simulink model "sm_car"  (R2025a)
settings: Solver=ode23t  StartTime=0.0  StopTime=400  MaxStep=0.4  RelTol=1e-3  AbsTol=1e-3  EnableMultiTasking=on
PreLoadFcn:
  | % Due to usability issue in Repeating Sequence block
  | warning('off','Simulink:Masking:Invalid');
  | 
  | % Eliminate unnecessary warnings in inactive variants
  | % Warnings generated only if you click through inactive variant
  | warning('off','MATLAB:nonExistentField');
  | warning('off','Simulink:Parameters:BlkParamUndefined');
PostLoadFcn:
  | set_param([bdroot '/Vehicle'],'popup_trailer','Off')
  | warning('off','sm:sli:setup:compile:LocalSolverNotSupported')
  | %sm_car_config_maneuver(bdroot,'WOT Braking');
  | sm_car_config_vehicle(bdroot,'false');
  | sm_car_config_logging(bdroot);
InitFcn:
  | sm_car_config_camera;
  | Vehicle = sm_car_vehcfg_checkConfig(Vehicle);
  | sm_car_check_tire_model(bdroot);
StartFcn:
  | tic;
StopFcn:
  | Elapsed_Sim_Time = toc;
  | % disp(['Elapsed Sim Time = ' num2str(Elapsed_Sim_Time)]);
undefined symbols (not defined in the file): Axle1D, AxleIn, Camera, Control, Driver, Free, Init, Maneuver, Pedal, RaceFix, RaceSpin, Scene, ShaftL1, ShaftL2, ShaftR1, ShaftR2, Soft, Stiff, Visual, X, xy_data_car_side, Y, Z
libraries: sm_lib x1546, nesl_utility x528, fl_lib x480, SimscapeFluids_lib x61, sdl_lib x49, simulink x29, ee_lib x7, simulink_extras x6, Linkage_Systems x4, Tire_1x2x x4, AntiRollBar_Systems x2, Linkage_Decoupled x2
(part 17 of 79)

== system sm_car/Vehicle/Vehicle/Chassis/Spring/Decoupled/Spring A1 Heave ==
  "Ctrl " : Inport
  AirOilPiston : Subsystem  VariantControl=AirOilPiston  mask(Hydropneumatic Spring Damper with Ride Height Control){spr_hp_top=Spring.sTop.Value, spr_hp_bot=Spring.sBottom.Value, t_ambient=Spring.Spring.TAmbient.Value, gspr_gas_properties=Spring.Spring.GasProperties, strut_oil_properties=Spring.Strut.OilProperties, gas_chamber_soft_area=Spring.Spring.GasSoft.A.Value, gas_chamber_stiff_area=Spring.Spring.GasStiff.A.Value, gas_chamber_soft_deadvol=Spring.Spring.GasSoft.volDead.Value, gas_chamber_stiff_deadvol=Spring.Spring.GasStiff.volDead.Value, gspr_mass_soft=Spring.Spring.GasSoft.mPiston.Value, gspr_mass_stiff=Spring.Spring.GasStiff.mPiston.Value, gspr_damping_soft=Spring.Spring.GasSoft.b.Value, gspr_damping_stiff=Spring.Spring.GasStiff.b.Value, gas_chamber_soft_x0=Spring.Spring.GasSoft.xInit.Value, gas_chamber_stiff_x0=Spring.Spring.GasStiff.xInit.Value, gas_chamber_soft_p0=Spring.Spring.GasSoft.pInit.Value, gas_chamber_stiff_p0=Spring.Spring.GasStiff.pInit.Value, gspr_cwall_soft=Spring.Spring.GasSoft.CWall.Value, gspr_cwall_stiff=Spring.Spring.GasStiff.CWall.Value, oil_chamber_soft_area=Spring.Spring.OilSoft.A.Value, oil_chamber_stiff_area=Spring.Spring.OilStiff.A.Value, oil_chamber_soft_deadvol=Spring.Spring.OilSoft.volDead.Value, oil_chamber_stiff_deadvol=Spring.Spring.OilStiff.volDead.Value, oil_chamber_soft_x0=Spring.Spring.OilSoft.xInit.Value, oil_chamber_stiff_x0=Spring.Spring.OilStiff.xInit.Value, oil_chamber_soft_p0=Spring.Spring.OilSoft.pInit.Value, oil_chamber_stiff_p0=Spring.Spring.OilStiff.pInit.Value, gsprv_smax_soft=Spring.Spring.ValveSoft.xMaxOpen.Value, gsprv_smax_stiff=Spring.Spring.ValveStiff.xMaxOpen.Value, gsprv_delsmax_soft=Spring.Spring.ValveSoft.xCloseToOpen.Value, gsprv_delsmax_stiff=Spring.Spring.ValveStiff.xCloseToOpen.Value, gsprv_arealeak_soft=Spring.Spring.ValveSoft.areaLeak.Value, gsprv_arealeak_stiff=Spring.Spring.ValveStiff.areaLeak.Value, gsprv_areamax_soft=Spring.Spring.ValveSoft.aMax.Value, gsprv_areamax_stiff=Spring.Spring.ValveStiff.aMax.Value, gsprv_cd_soft=Spring.Spring.ValveSoft.Cd.Value, gsprv_cd_stiff=Spring.Spring.ValveStiff.Cd.Value, gsprv_smooth_soft=Spring.Spring.ValveSoft.smoothFactor.Value, gsprv_smooth_stiff=Spring.Spring.ValveStiff.smoothFactor.Value, gsprva_stroke_soft=Spring.Spring.ValveActuatorSoft.xStroke.Value, gsprva_stroke_stiff=Spring.Spring.ValveActuatorStiff.xStroke.Value, gsprva_ton_soft=Spring.Spring.ValveActuatorSoft.tOn.Value, gsprva_ton_stiff=Spring.Spring.ValveActuatorStiff.tOn.Value, gsprva_toff_soft=Spring.Spring.ValveActuatorSoft.tOff.Value, gsprva_toff_stiff=Spring.Spring.ValveActuatorStiff.tOff.Value, strut_deadvol=Spring.Strut.volDead.Value, strut_area=Spring.Strut.A.Value, strut_x0=Spring.Strut.xInit.Value, strut_frc_colfrc=Spring.Strut.Friction.fCoulomb.Value, strut_frc_brkfrc=Spring.Strut.Friction.fBreakaway.Value, strut_frc_brkvel=Spring.Strut.Friction.vBreakaway.Value, strut_frc_visccoeff=Spring.Strut.Friction.mu.Value, bs_lim_upper=Spring.Endstop.xMax.Value, bs_lim_lower=Spring.Endstop.xMin.Value, bs_k_upper=Spring.Endstop.KxMax.Value, bs_k_lower=Spring.Endstop.KxMin.Value, bs_b_upper=Spring.Endstop.dxMax.Value, bs_b_lower=Spring.Endstop.dxMin.Value, bs_region=Spring.Endstop.xTransition.Value, p_diff_TLU_constant=Spring.Damper.Orifice.pDiff.Value, vol_flow_TLU_constant=Spring.Damper.Orifice.q.Value, dpr_restrarea_comp=Spring.Damper.RestrictionComp.A.Value, dpr_restrarea_reb=Spring.Damper.RestrictionReb.A.Value, dpr_cd_comp=Spring.Damper.RestrictionComp.Cd.Value, dpr_cd_reb=Spring.Damper.RestrictionReb.Cd.Value, dpr_prv_psetdiff_comp=Spring.Damper.PRVComp.pDiff.Value, dpr_prv_psetdiff_reb=Spring.Damper.PRVReb.pDiff.Value, dpr_prv_prange_comp=Spring.Damper.PRVComp.pRange.Value, dpr_prv_prange_reb=Spring.Damper.PRVReb.pRange.Value, dpr_prv_areamax_comp=Spring.Damper.PRVComp.A.Value, dpr_prv_areamax_reb=Spring.Damper.PRVReb.A.Value, dpr_prv_cd_comp=Spring.Damper.PRVComp.Cd.Value, dpr_prv_cd_reb=Spring.Damper.PRVReb.Cd.Value, dpr_cvdvalve_cmpos=Spring.CVDValve.Orifice.x.Value, dpr_cvdvalve_orifice_area=Spring.CVDValve.Orifice.A.Value, dpr_cvdvalve_orifice_pdiff=Spring.CVDValve.Orifice.pDiff.Value, dpr_cvdvalve_pcv_areamax=Spring.CVDValve.PCValve.AMax.Value, dpr_cvdvalve_pcv_prange=Spring.CVDValve.PCValve.pRange.Value, dpr_cvdvalve_arealeak=Spring.CVDValve.PCValve.ALeak.Value, dpr_cvdvalve_cd=Spring.CVDValve.PCValve.Cd.Value, dpr_cvdvalve_act_ts=Spring.CVDValve.tFilt.Value, rh_srcpressure=Spring.RideHeight.pSource.Value, rh_fcv_cmpos_inlet=Spring.RideHeight.OrificeInlet.x.Value, rh_fcv_cmpos_outlet=Spring.RideHeight.OrificeOutlet.x.Value, rh_fcv_orificearea_inlet=Spring.RideHeight.OrificeInlet.A.Value, rh_fcv_orificearea_outlet=Spring.RideHeight.OrificeOutlet.A.Value, rh_fcv_orificepdiff_inlet=Spring.RideHeight.OrificeInlet.pDiff.Value, rh_fcv_orificepdiff_outlet=Spring.RideHeight.OrificeOutlet.pDiff.Value, rh_fcv_pcprange_inlet=Spring.RideHeight.PCValveInlet.pRange.Value, rh_fcv_pcprange_outlet=Spring.RideHeight.PCValveOutlet.pRange.Value, rh_fcv_pcamax_inlet=Spring.RideHeight.PCValveInlet.AMax.Value, rh_fcv_pcamax_outlet=Spring.RideHeight.PCValveOutlet.AMax.Value, rh_fcv_arealeak_inlet=Spring.RideHeight.PCValveInlet.ALeak.Value, rh_fcv_arealeak_outlet=Spring.RideHeight.PCValveOutlet.ALeak.Value, rh_fcv_cd_inlet=Spring.RideHeight.PCValveInlet.Cd.Value, rh_fcv_cd_outlet=Spring.RideHeight.PCValveOutlet.Cd.Value, rh_fcv_smooth_inlet=Spring.RideHeight.PCValveInlet.smoothFactor.Value, rh_fcv_smooth_outlet=Spring.RideHeight.PCValveOutlet.smoothFactor.Value, rh_fcv_tfilt_inlet=Spring.RideHeight.PCValveInlet.tFilt.Value, rh_fcv_tfilt_outlet=Spring.RideHeight.PCValveOutlet.tFilt.Value}
      mask prompts: spr_hp_top "HP Top (m)"; spr_hp_bot "HP Bottom (m)"; t_ambient "Ambient Temperature (K)"; gspr_gas_properties "Gas Properties"; strut_oil_properties "Oil Properties"; strut_deadvol "Dead Volume (l)"; strut_area "Area (m^2)"; strut_x0 "Initial Disp. (m)"; strut_frc_colfrc "Coulomb Friction (N)"; strut_frc_brkfrc "Breakaway Force (N)"; strut_frc_brkvel "Breakaway Vel (m/s)"; strut_frc_visccoeff "Viscous Friction (N/(m/s))"; bs_region "Transition Region (m)"; p_diff_TLU_constant "Pressure Drop Vector (MPa)"; vol_flow_TLU_constant "Vol Flow Rate (m^3/s)"; dpr_cvdvalve_cmpos "Orifice Pos. Vector (m)"; dpr_cvdvalve_orifice_area "Orifice Area (m^2)"; dpr_cvdvalve_orifice_pdiff "Orifice Set Press. Diff. (bar)"; dpr_cvdvalve_pcv_areamax "Pr. Comp. Valve Max Area (m^2)"; dpr_cvdvalve_pcv_prange "Pr. Comp. Valve Range (bar)"; dpr_cvdvalve_arealeak "Leakage Area (m^2)"; dpr_cvdvalve_cd "Discharge Coeff (Cd)"; dpr_cvdvalve_act_ts "Actuator Time Constant (s)"; rh_srcpressure "Source Pressure (MPa)"
      mask help: Hydropneumatic spring damper with ride height control. Control signal selects soft or stiff gas spring. Damper has unique rebound and compression characteristics. Ride height can be raised or lowered.
      mask init:
      | spr_len0 = norm(spr_hp_top-spr_hp_bot);
      | 
      | gasprop_R  = gspr_gas_properties.R.Value;
      | gasprop_h  = gspr_gas_properties.h.Value;
      | gasprop_cp = gspr_gas_properties.cp.Value;
      | gasprop_mu = gspr_gas_properties.mu.Value;
      | gasprop_k  = gspr_gas_properties.k.Value;
      | 
      | oilprop_rho = strut_oil_properties.rho.Value;
      | oilprop_B   = strut_oil_properties.B.Value;
      | oilprop_nu  = strut_oil_properties.nu.Value;
      mask TypeOptions t_ambient: Ambient/temperature
      mask TypeOptions gas_chamber_soft_area:
      | Chamber
      | Gas Spring
      | Soft/interface_area
      mask TypeOptions gas_chamber_stiff_area:
      | Chamber
      | Gas Spring
      | Stiff/interface_area
      mask TypeOptions gas_chamber_soft_deadvol:
      | Chamber
      | Gas Spring
      | Soft/dead_volume
      mask TypeOptions gas_chamber_stiff_deadvol:
      | Chamber
      | Gas Spring
      | Stiff/dead_volume
      mask TypeOptions gspr_mass_soft:
      | Mass
      | Gas Spring
      | Soft/mass
      mask TypeOptions gspr_mass_stiff:
      | Mass
      | Gas Spring
      | Stiff/mass
      mask TypeOptions gspr_damping_soft:
      | Damper
      | Gas
      | Spring
      | Soft/D
      mask TypeOptions gspr_damping_stiff:
      | Damper
      | Gas
      | Spring
      | Stiff
      | /D
      mask TypeOptions gas_chamber_soft_x0:
      | Chamber
      | Gas Spring
      | Soft/length_init
      mask TypeOptions gas_chamber_stiff_x0:
      | Chamber
      | Gas Spring
      | Stiff/length_init
      mask TypeOptions gas_chamber_soft_p0:
      | Chamber
      | Gas Spring
      | Soft/p_I
      mask TypeOptions gas_chamber_stiff_p0:
      | Chamber
      | Gas Spring
      | Stiff/p_I
      mask TypeOptions gspr_cwall_soft: ThermResGasSoft/resistance
      mask TypeOptions gspr_cwall_stiff: ThermResGasStiff/resistance
      mask TypeOptions oil_chamber_soft_area:
      | Chamber
      | Oil Soft/interface_area
      mask TypeOptions oil_chamber_stiff_area:
      | Chamber
      | Oil Stiff/interface_area
      mask TypeOptions oil_chamber_soft_deadvol:
      | Chamber
      | Oil Soft/dead_volume
      mask TypeOptions oil_chamber_stiff_deadvol:
      | Chamber
      | Oil Stiff/dead_volume
      mask TypeOptions oil_chamber_soft_x0:
      | Chamber
      | Oil Soft/x0
      mask TypeOptions oil_chamber_stiff_x0:
      | Chamber
      | Oil Stiff/x0
      mask TypeOptions oil_chamber_soft_p0:
      | Chamber
      | Oil Soft/p0
      mask TypeOptions oil_chamber_stiff_p0:
      | Chamber
      | Oil Stiff/p0
      mask TypeOptions gsprv_smax_soft:
      | Valve Soft
      | SV10-24 NC/S_max
      mask TypeOptions gsprv_smax_stiff:
      | Valve Stiff
      | SV10-25 NO/S_max
      mask TypeOptions gsprv_delsmax_soft:
      | Valve Soft
      | SV10-24 NC/del_S_max
      mask TypeOptions gsprv_delsmax_stiff:
      | Valve Stiff
      | SV10-25 NO/del_S_max
      mask TypeOptions gsprv_arealeak_soft:
      | Valve Soft
      | SV10-24 NC/area_leak
      mask TypeOptions gsprv_arealeak_stiff:
      | Valve Stiff
      | SV10-25 NO/area_leak
      mask TypeOptions gsprv_areamax_soft:
      | Valve Soft
      | SV10-24 NC/area_max
      mask TypeOptions gsprv_areamax_stiff:
      | Valve Stiff
      | SV10-25 NO/area_max
      mask TypeOptions gsprv_cd_soft:
      | Valve Soft
      | SV10-24 NC/Cd
      mask TypeOptions gsprv_cd_stiff:
      | Valve Stiff
      | SV10-25 NO/Cd
      mask TypeOptions gsprv_smooth_soft:
      | Valve Soft
      | SV10-24 NC/smoothing_factor
      mask TypeOptions gsprv_smooth_stiff:
      | Valve Stiff
      | SV10-25 NO/smoothing_factor
      mask TypeOptions gsprva_stroke_soft:
      | Valve Actuator
      | Spring Soft/stroke
      mask TypeOptions gsprva_stroke_stiff:
      | Valve Actuator
      | Spring Stiff/stroke
      mask TypeOptions gsprva_ton_soft:
      | Valve Actuator
      | Spring Soft/t_on
      mask TypeOptions gsprva_ton_stiff:
      | Valve Actuator
      | Spring Stiff/t_on
      mask TypeOptions gsprva_toff_soft:
      | Valve Actuator
      | Spring Soft/t_off
      mask TypeOptions gsprva_toff_stiff:
      | Valve Actuator
      | Spring Stiff/t_off
      mask TypeOptions strut_deadvol:
      | Chamber
      | Strut/dead_volume
      mask TypeOptions strut_area:
      | Chamber
      | Strut/interface_area
      mask TypeOptions strut_x0:
      | Chamber
      | Strut/x0
      mask TypeOptions strut_frc_colfrc:
      | Strut
      | Friction/Col_frc
      mask TypeOptions strut_frc_brkfrc:
      | Strut
      | Friction/brkwy_frc
      mask TypeOptions strut_frc_brkvel:
      | Strut
      | Friction/brkwy_vel
      mask TypeOptions strut_frc_visccoeff:
      | Strut
      | Friction/visc_coef
      mask TypeOptions bs_lim_upper:
      | Strut
      | Hard
      | Stop/upper_bnd
      mask TypeOptions bs_lim_lower:
      | Strut
      | Hard
      | Stop/lower_bnd
      mask TypeOptions bs_k_upper:
      | Strut
      | Hard
      | Stop/stiff_up
      mask TypeOptions bs_k_lower:
      | Strut
      | Hard
      | Stop/stiff_low
      mask TypeOptions bs_b_upper:
      | Strut
      | Hard
      | Stop/D_up
      mask TypeOptions bs_b_lower:
      | Strut
      | Hard
      | Stop/D_low
      mask TypeOptions bs_region:
      | Strut
      | Hard
      | Stop/transition
      mask TypeOptions p_diff_TLU_constant: Damper/p_diff_TLU_constant
      mask TypeOptions vol_flow_TLU_constant: Damper/vol_flow_TLU_constant
      mask TypeOptions dpr_restrarea_comp: Damper/dpr_restrarea_comp
      mask TypeOptions dpr_restrarea_reb: Damper/dpr_restrarea_reb
      mask TypeOptions dpr_cd_comp: Damper/dpr_cd_comp
      mask TypeOptions dpr_cd_reb: Damper/dpr_cd_reb
      mask TypeOptions dpr_prv_psetdiff_comp: Damper/dpr_prv_psetdiff_comp
      mask TypeOptions dpr_prv_psetdiff_reb: Damper/dpr_prv_psetdiff_reb
      mask TypeOptions dpr_prv_prange_comp: Damper/dpr_prv_prange_comp
      mask TypeOptions dpr_prv_prange_reb: Damper/dpr_prv_prange_reb
      mask TypeOptions dpr_prv_areamax_comp: Damper/dpr_prv_areamax_comp
      mask TypeOptions dpr_prv_areamax_reb: Damper/dpr_prv_areamax_reb
      mask TypeOptions dpr_prv_cd_comp: Damper/dpr_prv_cd_comp
      mask TypeOptions dpr_prv_cd_reb: Damper/dpr_prv_cd_reb
      mask TypeOptions dpr_cvdvalve_cmpos: Damper/dpr_cvdvalve_cmpos
      mask TypeOptions dpr_cvdvalve_orifice_area: Damper/dpr_cvdvalve_orifice_area
      mask TypeOptions dpr_cvdvalve_orifice_pdiff: Damper/dpr_cvdvalve_orifice_pdiff
      mask TypeOptions dpr_cvdvalve_pcv_areamax: Damper/dpr_cvdvalve_pcv_areamax
      mask TypeOptions dpr_cvdvalve_pcv_prange: Damper/dpr_cvdvalve_pcv_prange
      mask TypeOptions dpr_cvdvalve_arealeak: Damper/dpr_cvdvalve_arealeak
      mask TypeOptions dpr_cvdvalve_cd: Damper/dpr_cvdvalve_cd
      mask TypeOptions dpr_cvdvalve_act_ts: Damper/dpr_cvdvalve_act_ts
      mask TypeOptions rh_srcpressure: Ride Height/rh_srcpressure
      mask TypeOptions rh_fcv_cmpos_inlet: Ride Height/rh_fcv_cmpos_inlet
      mask TypeOptions rh_fcv_cmpos_outlet: Ride Height/rh_fcv_cmpos_outlet
      mask TypeOptions rh_fcv_orificearea_inlet: Ride Height/rh_fcv_orificearea_inlet
      mask TypeOptions rh_fcv_orificearea_outlet: Ride Height/rh_fcv_orificearea_outlet
      mask TypeOptions rh_fcv_orificepdiff_inlet: Ride Height/rh_fcv_orificepdiff_inlet
      mask TypeOptions rh_fcv_orificepdiff_outlet: Ride Height/rh_fcv_orificepdiff_outlet
      mask TypeOptions rh_fcv_pcprange_inlet: Ride Height/rh_fcv_pcprange_inlet
      mask TypeOptions rh_fcv_pcprange_outlet: Ride Height/rh_fcv_pcprange_outlet
      mask TypeOptions rh_fcv_pcamax_inlet: Ride Height/rh_fcv_pcamax_inlet
      mask TypeOptions rh_fcv_pcamax_outlet: Ride Height/rh_fcv_pcamax_outlet
      mask TypeOptions rh_fcv_arealeak_inlet: Ride Height/rh_fcv_arealeak_inlet
      mask TypeOptions rh_fcv_arealeak_outlet: Ride Height/rh_fcv_arealeak_outlet
      mask TypeOptions rh_fcv_cd_inlet: Ride Height/rh_fcv_cd_inlet
      mask TypeOptions rh_fcv_cd_outlet: Ride Height/rh_fcv_cd_outlet
      mask TypeOptions rh_fcv_smooth_inlet: Ride Height/rh_fcv_smooth_inlet
      mask TypeOptions rh_fcv_smooth_outlet: Ride Height/rh_fcv_smooth_outlet
      mask TypeOptions rh_fcv_tfilt_inlet: Ride Height/rh_fcv_tfilt_inlet
      mask TypeOptions rh_fcv_tfilt_outlet: Ride Height/rh_fcv_tfilt_outlet
      mask DialogControl tab_gas_spring Prompt: Gas Spring
      mask DialogControl cont_gas_spring_gas Prompt: Gas Side
      mask DialogControl text_gspr_soft Prompt: Soft
      mask DialogControl text_gspr_stiff Prompt: Stiff
      mask DialogControl text_gspr_area Prompt: Area (m^2)
      mask DialogControl text_gspr_deadvol Prompt: Dead Volume (l)
      mask DialogControl text_gspr_pistmass Prompt: Piston Mass (kg)
      mask DialogControl text_gspr_damping Prompt: Damping (N/(m/s))
      mask DialogControl text_gspr_x0 Prompt: Initial Disp. (m)
      mask DialogControl text_gspr_p0 Prompt: Initial Press. (MPa)
      mask DialogControl text_gspr_cwall Prompt: Wall (K/W)
      mask DialogControl cont_gas_spring_oil Prompt: Oil Side
      mask DialogControl text_gspro_soft Prompt: Soft
      mask DialogControl text_gspro_stiff Prompt: Stiff
      mask DialogControl text_gspro_area Prompt: Area (m^2)
      mask DialogControl text_gspro_deadvol Prompt: Dead Volume (l)
      mask DialogControl text_gspro_x0 Prompt: Initial Disp. (m)
      mask DialogControl text_oil_chamber_x0 Prompt: Initial Press. (MPa)
      mask DialogControl cont_gas_spring_valve Prompt: Valve
      mask DialogControl text_gsprv_soft Prompt: Soft
      mask DialogControl text_gsprv_stiff Prompt: Stiff
      mask DialogControl text_gsprv_xopen Prompt: Travel at Open (m)
      mask DialogControl text_gsprv_delSmax Prompt: Closed to Open (m)
      mask DialogControl text_gsprv_areaLeak Prompt: Leakage (m^2)
      mask DialogControl text_gsprv_areaMax Prompt: Area Max (m^2)
      mask DialogControl text_gsprv_cd Prompt: Cd
      mask DialogControl text_gsprv_smooth Prompt: Smooth
      mask DialogControl cont_gas_spring_valveact Prompt: Valve Actuator
      mask DialogControl text_gsprva_soft Prompt: Soft
      mask DialogControl text_gsprva_stiff Prompt: Stiff
      mask DialogControl text_gsprva_stroke Prompt: Stroke (m)
      mask DialogControl text_gsprva_ton Prompt: On Time (s)
      mask DialogControl text_gsprva_toff Prompt: Off Time (s)
      mask DialogControl cont_oil_strut Prompt: Strut
      mask DialogControl cont_endstop Prompt: Endstop
      mask DialogControl text_endstop_upper Prompt: Upper
      mask DialogControl text_endstop_lower Prompt: Lower
      mask DialogControl text_endstop_limit Prompt: Limit (m)
      mask DialogControl text_endstop_stiffness Prompt: Stiffness (N/m)
      mask DialogControl text_endstop_damping Prompt: Damping (N/(m/s))
      mask DialogControl tab_damper Prompt: Damper
      mask DialogControl cont_orifice_ls Prompt: Low Speed Orifice
      mask DialogControl cont_blowoff_restriction Prompt: Blowoff Restriction
      mask DialogControl text_blowoff_comp Prompt: Compression
      mask DialogControl text_blowoff_reb Prompt: Rebound
      mask DialogControl text_restr_area Prompt: Restr. Area (m^2)
      mask DialogControl text_cd Prompt: Cd
      mask DialogControl cont_blowoff_prv Prompt: Blowoff PRV
      mask DialogControl text_blowoff_prv_comp Prompt: Compression
      mask DialogControl text_blowoff_prv_reb Prompt: Rebound
      mask DialogControl text_psetdiff Prompt: Press. Diff. (MPa)
      mask DialogControl text_prange Prompt: Press. Range (MPa)
      mask DialogControl text_areamax Prompt: Max Area (m^2)
      mask DialogControl text_blowoff_cd Prompt: Cd
      mask DialogControl cont_dpr_cvd_valve Prompt: CVD Valve
      mask DialogControl tab_ride_height Prompt: Ride Height
      mask DialogControl text_rideheight_inlet Prompt: Inlet
      mask DialogControl text_rideheight_outlet Prompt: Outlet
      mask DialogControl text_rh_prcv_cmpos Prompt: Orifice Pos. Vec. (m)
      mask DialogControl text_rh_prcv_orificearea Prompt: Orifice Area Vec (m^2)
      mask DialogControl text_rh_prcv_orificepdiff Prompt: Orifice Pr. Diff (bar)
      mask DialogControl text_rh_prcv_pcprange Prompt: Pr. Comp. Range (bar)
      mask DialogControl text_rh_prcv_pcamax Prompt: Pr. Comp. A Max (m^2)
      mask DialogControl text_rh_prcv_arealeak Prompt: Leakage Area (m^2)
      mask DialogControl text_rh_prcv_cd Prompt: Cd
      mask DialogControl text_rh_fcv_smooth Prompt: Smoothing
      mask DialogControl text_rh_fcv_tfilt Prompt: Time Constant (s)
  Linear : Subsystem  VariantControl=Linear  mask(Linear Spring){spr_def0=Spring.xPreload.Value, spr_frc0=Spring.fPreload.Value, spr_k=Spring.K.Value, spr_hp_top=Spring.sTop.Value, spr_hp_bot=Spring.sBottom.Value}
      mask prompts: spr_def0 "Preload Deformation (m)"; spr_frc0 "Preload Force (N)"; spr_k "Spring Rate (N/m)"; spr_hp_top "HP Top [xyz] (m)"; spr_hp_bot "HP Bottom [xyz] (m)"
      mask help: Spring with linear stiffness. Preload can be specified using deformation or force, unused value must be zero. If both are non-zero, preload deformation is used.
      mask init:
      | spr_len0 = norm(spr_hp_top-spr_hp_bot);
      | 
      | curblk = gcb;
      | if(abs(spr_def0)>0)
      | set_param([curblk '/Spring'],...
      |     'f_specify','Off',...
      |     'x_priority','High');
      | else
      | set_param([curblk '/Spring'],...
      |     'f_specify','On',...
      |     'x_priority','None');
      | end
      mask DialogControl Container3 Prompt: Specify Preload Deformation or Force, other value is 0
  No Spring : Subsystem  VariantControl=No_Spring  mask(No Spring){}
      mask help: Sensor only
  Nonlinear : Subsystem  VariantControl=Nonlinear  mask(Nonlinear Spring){spr_def0=Spring.xPreload.Value, spr_frc0=Spring.fPreload.Value, deformation_vector=Spring.xSpring.Value, force_vector=Spring.fSpring.Value, spr_hp_top=Spring.sTop.Value, spr_hp_bot=Spring.sBottom.Value}
      mask prompts: spr_def0 "Preload Deformation (m)"; spr_frc0 "Preload Force (N)"; deformation_vector "Deformation vector"; force_vector "Force vector"; spr_hp_top "HP Top [xyz] (m)"; spr_hp_bot "HP Bottom [xyz] (m)"
      mask help: Spring with stiffness specified by a lookup table. Preload can be specified using deformation or force, unused value must be zero. If both are non-zero, preload deformation is used.
      mask init:
      | spr_len0 = norm(spr_hp_top-spr_hp_bot);
      | 
      | curblk = gcb;
      | spr_x0 = -spr_def0;
      | if(spr_def0==0 && (abs(spr_frc0)>0))
      | spr_x0 = -interp1(force_vector,deformation_vector,spr_frc0);
      | end
      mask TypeOptions deformation_vector: Spring/deformation_vector
      mask TypeOptions force_vector: Spring/force_vector
      mask DialogControl Container3 Prompt: Specify Preload Deformation or Force, other value is 0
  " R" : PMIOPort  Side=Left
  " C" : PMIOPort  Port=2  Side=Right
  " meas" : Outport  VectorParamsAs1DForOutWhenUnconnected=off

== system sm_car/Vehicle/Vehicle/Chassis/Spring/Decoupled/Spring A1 Roll ==
  "Ctrl " : Inport
  AirOilPiston : Subsystem  VariantControl=AirOilPiston  mask(Hydropneumatic Spring Damper with Ride Height Control){spr_hp_top=Spring.sTop.Value, spr_hp_bot=Spring.sBottom.Value, t_ambient=Spring.Spring.TAmbient.Value, gspr_gas_properties=Spring.Spring.GasProperties, strut_oil_properties=Spring.Strut.OilProperties, gas_chamber_soft_area=Spring.Spring.GasSoft.A.Value, gas_chamber_stiff_area=Spring.Spring.GasStiff.A.Value, gas_chamber_soft_deadvol=Spring.Spring.GasSoft.volDead.Value, gas_chamber_stiff_deadvol=Spring.Spring.GasStiff.volDead.Value, gspr_mass_soft=Spring.Spring.GasSoft.mPiston.Value, gspr_mass_stiff=Spring.Spring.GasStiff.mPiston.Value, gspr_damping_soft=Spring.Spring.GasSoft.b.Value, gspr_damping_stiff=Spring.Spring.GasStiff.b.Value, gas_chamber_soft_x0=Spring.Spring.GasSoft.xInit.Value, gas_chamber_stiff_x0=Spring.Spring.GasStiff.xInit.Value, gas_chamber_soft_p0=Spring.Spring.GasSoft.pInit.Value, gas_chamber_stiff_p0=Spring.Spring.GasStiff.pInit.Value, gspr_cwall_soft=Spring.Spring.GasSoft.CWall.Value, gspr_cwall_stiff=Spring.Spring.GasStiff.CWall.Value, oil_chamber_soft_area=Spring.Spring.OilSoft.A.Value, oil_chamber_stiff_area=Spring.Spring.OilStiff.A.Value, oil_chamber_soft_deadvol=Spring.Spring.OilSoft.volDead.Value, oil_chamber_stiff_deadvol=Spring.Spring.OilStiff.volDead.Value, oil_chamber_soft_x0=Spring.Spring.OilSoft.xInit.Value, oil_chamber_stiff_x0=Spring.Spring.OilStiff.xInit.Value, oil_chamber_soft_p0=Spring.Spring.OilSoft.pInit.Value, oil_chamber_stiff_p0=Spring.Spring.OilStiff.pInit.Value, gsprv_smax_soft=Spring.Spring.ValveSoft.xMaxOpen.Value, gsprv_smax_stiff=Spring.Spring.ValveStiff.xMaxOpen.Value, gsprv_delsmax_soft=Spring.Spring.ValveSoft.xCloseToOpen.Value, gsprv_delsmax_stiff=Spring.Spring.ValveStiff.xCloseToOpen.Value, gsprv_arealeak_soft=Spring.Spring.ValveSoft.areaLeak.Value, gsprv_arealeak_stiff=Spring.Spring.ValveStiff.areaLeak.Value, gsprv_areamax_soft=Spring.Spring.ValveSoft.aMax.Value, gsprv_areamax_stiff=Spring.Spring.ValveStiff.aMax.Value, gsprv_cd_soft=Spring.Spring.ValveSoft.Cd.Value, gsprv_cd_stiff=Spring.Spring.ValveStiff.Cd.Value, gsprv_smooth_soft=Spring.Spring.ValveSoft.smoothFactor.Value, gsprv_smooth_stiff=Spring.Spring.ValveStiff.smoothFactor.Value, gsprva_stroke_soft=Spring.Spring.ValveActuatorSoft.xStroke.Value, gsprva_stroke_stiff=Spring.Spring.ValveActuatorStiff.xStroke.Value, gsprva_ton_soft=Spring.Spring.ValveActuatorSoft.tOn.Value, gsprva_ton_stiff=Spring.Spring.ValveActuatorStiff.tOn.Value, gsprva_toff_soft=Spring.Spring.ValveActuatorSoft.tOff.Value, gsprva_toff_stiff=Spring.Spring.ValveActuatorStiff.tOff.Value, strut_deadvol=Spring.Strut.volDead.Value, strut_area=Spring.Strut.A.Value, strut_x0=Spring.Strut.xInit.Value, strut_frc_colfrc=Spring.Strut.Friction.fCoulomb.Value, strut_frc_brkfrc=Spring.Strut.Friction.fBreakaway.Value, strut_frc_brkvel=Spring.Strut.Friction.vBreakaway.Value, strut_frc_visccoeff=Spring.Strut.Friction.mu.Value, bs_lim_upper=Spring.Endstop.xMax.Value, bs_lim_lower=Spring.Endstop.xMin.Value, bs_k_upper=Spring.Endstop.KxMax.Value, bs_k_lower=Spring.Endstop.KxMin.Value, bs_b_upper=Spring.Endstop.dxMax.Value, bs_b_lower=Spring.Endstop.dxMin.Value, bs_region=Spring.Endstop.xTransition.Value, p_diff_TLU_constant=Spring.Damper.Orifice.pDiff.Value, vol_flow_TLU_constant=Spring.Damper.Orifice.q.Value, dpr_restrarea_comp=Spring.Damper.RestrictionComp.A.Value, dpr_restrarea_reb=Spring.Damper.RestrictionReb.A.Value, dpr_cd_comp=Spring.Damper.RestrictionComp.Cd.Value, dpr_cd_reb=Spring.Damper.RestrictionReb.Cd.Value, dpr_prv_psetdiff_comp=Spring.Damper.PRVComp.pDiff.Value, dpr_prv_psetdiff_reb=Spring.Damper.PRVReb.pDiff.Value, dpr_prv_prange_comp=Spring.Damper.PRVComp.pRange.Value, dpr_prv_prange_reb=Spring.Damper.PRVReb.pRange.Value, dpr_prv_areamax_comp=Spring.Damper.PRVComp.A.Value, dpr_prv_areamax_reb=Spring.Damper.PRVReb.A.Value, dpr_prv_cd_comp=Spring.Damper.PRVComp.Cd.Value, dpr_prv_cd_reb=Spring.Damper.PRVReb.Cd.Value, dpr_cvdvalve_cmpos=Spring.CVDValve.Orifice.x.Value, dpr_cvdvalve_orifice_area=Spring.CVDValve.Orifice.A.Value, dpr_cvdvalve_orifice_pdiff=Spring.CVDValve.Orifice.pDiff.Value, dpr_cvdvalve_pcv_areamax=Spring.CVDValve.PCValve.AMax.Value, dpr_cvdvalve_pcv_prange=Spring.CVDValve.PCValve.pRange.Value, dpr_cvdvalve_arealeak=Spring.CVDValve.PCValve.ALeak.Value, dpr_cvdvalve_cd=Spring.CVDValve.PCValve.Cd.Value, dpr_cvdvalve_act_ts=Spring.CVDValve.tFilt.Value, rh_srcpressure=Spring.RideHeight.pSource.Value, rh_fcv_cmpos_inlet=Spring.RideHeight.OrificeInlet.x.Value, rh_fcv_cmpos_outlet=Spring.RideHeight.OrificeOutlet.x.Value, rh_fcv_orificearea_inlet=Spring.RideHeight.OrificeInlet.A.Value, rh_fcv_orificearea_outlet=Spring.RideHeight.OrificeOutlet.A.Value, rh_fcv_orificepdiff_inlet=Spring.RideHeight.OrificeInlet.pDiff.Value, rh_fcv_orificepdiff_outlet=Spring.RideHeight.OrificeOutlet.pDiff.Value, rh_fcv_pcprange_inlet=Spring.RideHeight.PCValveInlet.pRange.Value, rh_fcv_pcprange_outlet=Spring.RideHeight.PCValveOutlet.pRange.Value, rh_fcv_pcamax_inlet=Spring.RideHeight.PCValveInlet.AMax.Value, rh_fcv_pcamax_outlet=Spring.RideHeight.PCValveOutlet.AMax.Value, rh_fcv_arealeak_inlet=Spring.RideHeight.PCValveInlet.ALeak.Value, rh_fcv_arealeak_outlet=Spring.RideHeight.PCValveOutlet.ALeak.Value, rh_fcv_cd_inlet=Spring.RideHeight.PCValveInlet.Cd.Value, rh_fcv_cd_outlet=Spring.RideHeight.PCValveOutlet.Cd.Value, rh_fcv_smooth_inlet=Spring.RideHeight.PCValveInlet.smoothFactor.Value, rh_fcv_smooth_outlet=Spring.RideHeight.PCValveOutlet.smoothFactor.Value, rh_fcv_tfilt_inlet=Spring.RideHeight.PCValveInlet.tFilt.Value, rh_fcv_tfilt_outlet=Spring.RideHeight.PCValveOutlet.tFilt.Value}
      mask prompts: spr_hp_top "HP Top (m)"; spr_hp_bot "HP Bottom (m)"; t_ambient "Ambient Temperature (K)"; gspr_gas_properties "Gas Properties"; strut_oil_properties "Oil Properties"; strut_deadvol "Dead Volume (l)"; strut_area "Area (m^2)"; strut_x0 "Initial Disp. (m)"; strut_frc_colfrc "Coulomb Friction (N)"; strut_frc_brkfrc "Breakaway Force (N)"; strut_frc_brkvel "Breakaway Vel (m/s)"; strut_frc_visccoeff "Viscous Friction (N/(m/s))"; bs_region "Transition Region (m)"; p_diff_TLU_constant "Pressure Drop Vector (MPa)"; vol_flow_TLU_constant "Vol Flow Rate (m^3/s)"; dpr_cvdvalve_cmpos "Orifice Pos. Vector (m)"; dpr_cvdvalve_orifice_area "Orifice Area (m^2)"; dpr_cvdvalve_orifice_pdiff "Orifice Set Press. Diff. (bar)"; dpr_cvdvalve_pcv_areamax "Pr. Comp. Valve Max Area (m^2)"; dpr_cvdvalve_pcv_prange "Pr. Comp. Valve Range (bar)"; dpr_cvdvalve_arealeak "Leakage Area (m^2)"; dpr_cvdvalve_cd "Discharge Coeff (Cd)"; dpr_cvdvalve_act_ts "Actuator Time Constant (s)"; rh_srcpressure "Source Pressure (MPa)"
      mask help: Hydropneumatic spring damper with ride height control. Control signal selects soft or stiff gas spring. Damper has unique rebound and compression characteristics. Ride height can be raised or lowered.
      mask init: same as sm_car/Vehicle/Vehicle/Chassis/Spring/Decoupled/Spring A1 Heave/AirOilPiston
      mask TypeOptions t_ambient: Ambient/temperature
      mask TypeOptions gas_chamber_soft_area:
      | Chamber
      | Gas Spring
      | Soft/interface_area
      mask TypeOptions gas_chamber_stiff_area:
      | Chamber
      | Gas Spring
      | Stiff/interface_area
      mask TypeOptions gas_chamber_soft_deadvol:
      | Chamber
      | Gas Spring
      | Soft/dead_volume
      mask TypeOptions gas_chamber_stiff_deadvol:
      | Chamber
      | Gas Spring
      | Stiff/dead_volume
      mask TypeOptions gspr_mass_soft:
      | Mass
      | Gas Spring
      | Soft/mass
      mask TypeOptions gspr_mass_stiff:
      | Mass
      | Gas Spring
      | Stiff/mass
      mask TypeOptions gspr_damping_soft:
      | Damper
      | Gas
      | Spring
      | Soft/D
      mask TypeOptions gspr_damping_stiff:
      | Damper
      | Gas
      | Spring
      | Stiff
      | /D
      mask TypeOptions gas_chamber_soft_x0:
      | Chamber
      | Gas Spring
      | Soft/length_init
      mask TypeOptions gas_chamber_stiff_x0:
      | Chamber
      | Gas Spring
      | Stiff/length_init
      mask TypeOptions gas_chamber_soft_p0:
      | Chamber
      | Gas Spring
      | Soft/p_I
      mask TypeOptions gas_chamber_stiff_p0:
      | Chamber
      | Gas Spring
      | Stiff/p_I
      mask TypeOptions gspr_cwall_soft: ThermResGasSoft/resistance
      mask TypeOptions gspr_cwall_stiff: ThermResGasStiff/resistance
      mask TypeOptions oil_chamber_soft_area:
      | Chamber
      | Oil Soft/interface_area
      mask TypeOptions oil_chamber_stiff_area:
      | Chamber
      | Oil Stiff/interface_area
      mask TypeOptions oil_chamber_soft_deadvol:
      | Chamber
      | Oil Soft/dead_volume
      mask TypeOptions oil_chamber_stiff_deadvol:
      | Chamber
      | Oil Stiff/dead_volume
      mask TypeOptions oil_chamber_soft_x0:
      | Chamber
      | Oil Soft/x0
      mask TypeOptions oil_chamber_stiff_x0:
      | Chamber
      | Oil Stiff/x0
      mask TypeOptions oil_chamber_soft_p0:
      | Chamber
      | Oil Soft/p0
      mask TypeOptions oil_chamber_stiff_p0:
      | Chamber
      | Oil Stiff/p0
      mask TypeOptions gsprv_smax_soft:
      | Valve Soft
      | SV10-24 NC/S_max
      mask TypeOptions gsprv_smax_stiff:
      | Valve Stiff
      | SV10-25 NO/S_max
      mask TypeOptions gsprv_delsmax_soft:
      | Valve Soft
      | SV10-24 NC/del_S_max
      mask TypeOptions gsprv_delsmax_stiff:
      | Valve Stiff
      | SV10-25 NO/del_S_max
      mask TypeOptions gsprv_arealeak_soft:
      | Valve Soft
      | SV10-24 NC/area_leak
      mask TypeOptions gsprv_arealeak_stiff:
      | Valve Stiff
      | SV10-25 NO/area_leak
      mask TypeOptions gsprv_areamax_soft:
      | Valve Soft
      | SV10-24 NC/area_max
      mask TypeOptions gsprv_areamax_stiff:
      | Valve Stiff
      | SV10-25 NO/area_max
      mask TypeOptions gsprv_cd_soft:
      | Valve Soft
      | SV10-24 NC/Cd
      mask TypeOptions gsprv_cd_stiff:
      | Valve Stiff
      | SV10-25 NO/Cd
      mask TypeOptions gsprv_smooth_soft:
      | Valve Soft
      | SV10-24 NC/smoothing_factor
      mask TypeOptions gsprv_smooth_stiff:
      | Valve Stiff
      | SV10-25 NO/smoothing_factor
      mask TypeOptions gsprva_stroke_soft:
      | Valve Actuator
      | Spring Soft/stroke
      mask TypeOptions gsprva_stroke_stiff:
      | Valve Actuator
      | Spring Stiff/stroke
      mask TypeOptions gsprva_ton_soft:
      | Valve Actuator
      | Spring Soft/t_on
      mask TypeOptions gsprva_ton_stiff:
      | Valve Actuator
      | Spring Stiff/t_on
      mask TypeOptions gsprva_toff_soft:
      | Valve Actuator
      | Spring Soft/t_off
      mask TypeOptions gsprva_toff_stiff:
      | Valve Actuator
      | Spring Stiff/t_off
      mask TypeOptions strut_deadvol:
      | Chamber
      | Strut/dead_volume
      mask TypeOptions strut_area:
      | Chamber
      | Strut/interface_area
      mask TypeOptions strut_x0:
      | Chamber
      | Strut/x0
      mask TypeOptions strut_frc_colfrc:
      | Strut
      | Friction/Col_frc
      mask TypeOptions strut_frc_brkfrc:
      | Strut
      | Friction/brkwy_frc
      mask TypeOptions strut_frc_brkvel:
      | Strut
      | Friction/brkwy_vel
      mask TypeOptions strut_frc_visccoeff:
      | Strut
      | Friction/visc_coef
      mask TypeOptions bs_lim_upper:
      | Strut
      | Hard
      | Stop/upper_bnd
      mask TypeOptions bs_lim_lower:
      | Strut
      | Hard
      | Stop/lower_bnd
      mask TypeOptions bs_k_upper:
      | Strut
      | Hard
      | Stop/stiff_up
      mask TypeOptions bs_k_lower:
      | Strut
      | Hard
      | Stop/stiff_low
      mask TypeOptions bs_b_upper:
      | Strut
      | Hard
      | Stop/D_up
      mask TypeOptions bs_b_lower:
      | Strut
      | Hard
      | Stop/D_low
      mask TypeOptions bs_region:
      | Strut
      | Hard
      | Stop/transition
      mask TypeOptions p_diff_TLU_constant: Damper/p_diff_TLU_constant
      mask TypeOptions vol_flow_TLU_constant: Damper/vol_flow_TLU_constant
      mask TypeOptions dpr_restrarea_comp: Damper/dpr_restrarea_comp
      mask TypeOptions dpr_restrarea_reb: Damper/dpr_restrarea_reb
      mask TypeOptions dpr_cd_comp: Damper/dpr_cd_comp
      mask TypeOptions dpr_cd_reb: Damper/dpr_cd_reb
      mask TypeOptions dpr_prv_psetdiff_comp: Damper/dpr_prv_psetdiff_comp
      mask TypeOptions dpr_prv_psetdiff_reb: Damper/dpr_prv_psetdiff_reb
      mask TypeOptions dpr_prv_prange_comp: Damper/dpr_prv_prange_comp
      mask TypeOptions dpr_prv_prange_reb: Damper/dpr_prv_prange_reb
      mask TypeOptions dpr_prv_areamax_comp: Damper/dpr_prv_areamax_comp
      mask TypeOptions dpr_prv_areamax_reb: Damper/dpr_prv_areamax_reb
      mask TypeOptions dpr_prv_cd_comp: Damper/dpr_prv_cd_comp
      mask TypeOptions dpr_prv_cd_reb: Damper/dpr_prv_cd_reb
      mask TypeOptions dpr_cvdvalve_cmpos: Damper/dpr_cvdvalve_cmpos
      mask TypeOptions dpr_cvdvalve_orifice_area: Damper/dpr_cvdvalve_orifice_area
      mask TypeOptions dpr_cvdvalve_orifice_pdiff: Damper/dpr_cvdvalve_orifice_pdiff
      mask TypeOptions dpr_cvdvalve_pcv_areamax: Damper/dpr_cvdvalve_pcv_areamax
      mask TypeOptions dpr_cvdvalve_pcv_prange: Damper/dpr_cvdvalve_pcv_prange
      mask TypeOptions dpr_cvdvalve_arealeak: Damper/dpr_cvdvalve_arealeak
      mask TypeOptions dpr_cvdvalve_cd: Damper/dpr_cvdvalve_cd
      mask TypeOptions dpr_cvdvalve_act_ts: Damper/dpr_cvdvalve_act_ts
      mask TypeOptions rh_srcpressure: Ride Height/rh_srcpressure
      mask TypeOptions rh_fcv_cmpos_inlet: Ride Height/rh_fcv_cmpos_inlet
      mask TypeOptions rh_fcv_cmpos_outlet: Ride Height/rh_fcv_cmpos_outlet
      mask TypeOptions rh_fcv_orificearea_inlet: Ride Height/rh_fcv_orificearea_inlet
      mask TypeOptions rh_fcv_orificearea_outlet: Ride Height/rh_fcv_orificearea_outlet
      mask TypeOptions rh_fcv_orificepdiff_inlet: Ride Height/rh_fcv_orificepdiff_inlet
      mask TypeOptions rh_fcv_orificepdiff_outlet: Ride Height/rh_fcv_orificepdiff_outlet
      mask TypeOptions rh_fcv_pcprange_inlet: Ride Height/rh_fcv_pcprange_inlet
      mask TypeOptions rh_fcv_pcprange_outlet: Ride Height/rh_fcv_pcprange_outlet
      mask TypeOptions rh_fcv_pcamax_inlet: Ride Height/rh_fcv_pcamax_inlet
      mask TypeOptions rh_fcv_pcamax_outlet: Ride Height/rh_fcv_pcamax_outlet
      mask TypeOptions rh_fcv_arealeak_inlet: Ride Height/rh_fcv_arealeak_inlet
      mask TypeOptions rh_fcv_arealeak_outlet: Ride Height/rh_fcv_arealeak_outlet
      mask TypeOptions rh_fcv_cd_inlet: Ride Height/rh_fcv_cd_inlet
      mask TypeOptions rh_fcv_cd_outlet: Ride Height/rh_fcv_cd_outlet
      mask TypeOptions rh_fcv_smooth_inlet: Ride Height/rh_fcv_smooth_inlet
      mask TypeOptions rh_fcv_smooth_outlet: Ride Height/rh_fcv_smooth_outlet
      mask TypeOptions rh_fcv_tfilt_inlet: Ride Height/rh_fcv_tfilt_inlet
      mask TypeOptions rh_fcv_tfilt_outlet: Ride Height/rh_fcv_tfilt_outlet
      mask DialogControl tab_gas_spring Prompt: Gas Spring
      mask DialogControl cont_gas_spring_gas Prompt: Gas Side
      mask DialogControl text_gspr_soft Prompt: Soft
      mask DialogControl text_gspr_stiff Prompt: Stiff
      mask DialogControl text_gspr_area Prompt: Area (m^2)
      mask DialogControl text_gspr_deadvol Prompt: Dead Volume (l)
      mask DialogControl text_gspr_pistmass Prompt: Piston Mass (kg)
      mask DialogControl text_gspr_damping Prompt: Damping (N/(m/s))
      mask DialogControl text_gspr_x0 Prompt: Initial Disp. (m)
      mask DialogControl text_gspr_p0 Prompt: Initial Press. (MPa)
      mask DialogControl text_gspr_cwall Prompt: Wall (K/W)
      mask DialogControl cont_gas_spring_oil Prompt: Oil Side
      mask DialogControl text_gspro_soft Prompt: Soft
      mask DialogControl text_gspro_stiff Prompt: Stiff
      mask DialogControl text_gspro_area Prompt: Area (m^2)
      mask DialogControl text_gspro_deadvol Prompt: Dead Volume (l)
      mask DialogControl text_gspro_x0 Prompt: Initial Disp. (m)
      mask DialogControl text_oil_chamber_x0 Prompt: Initial Press. (MPa)
      mask DialogControl cont_gas_spring_valve Prompt: Valve
      mask DialogControl text_gsprv_soft Prompt: Soft
      mask DialogControl text_gsprv_stiff Prompt: Stiff
      mask DialogControl text_gsprv_xopen Prompt: Travel at Open (m)
      mask DialogControl text_gsprv_delSmax Prompt: Closed to Open (m)
      mask DialogControl text_gsprv_areaLeak Prompt: Leakage (m^2)
      mask DialogControl text_gsprv_areaMax Prompt: Area Max (m^2)
      mask DialogControl text_gsprv_cd Prompt: Cd
      mask DialogControl text_gsprv_smooth Prompt: Smooth
      mask DialogControl cont_gas_spring_valveact Prompt: Valve Actuator
      mask DialogControl text_gsprva_soft Prompt: Soft
      mask DialogControl text_gsprva_stiff Prompt: Stiff
      mask DialogControl text_gsprva_stroke Prompt: Stroke (m)
      mask DialogControl text_gsprva_ton Prompt: On Time (s)
      mask DialogControl text_gsprva_toff Prompt: Off Time (s)
      mask DialogControl cont_oil_strut Prompt: Strut
      mask DialogControl cont_endstop Prompt: Endstop
      mask DialogControl text_endstop_upper Prompt: Upper
      mask DialogControl text_endstop_lower Prompt: Lower
      mask DialogControl text_endstop_limit Prompt: Limit (m)
      mask DialogControl text_endstop_stiffness Prompt: Stiffness (N/m)
      mask DialogControl text_endstop_damping Prompt: Damping (N/(m/s))
      mask DialogControl tab_damper Prompt: Damper
      mask DialogControl cont_orifice_ls Prompt: Low Speed Orifice
      mask DialogControl cont_blowoff_restriction Prompt: Blowoff Restriction
      mask DialogControl text_blowoff_comp Prompt: Compression
      mask DialogControl text_blowoff_reb Prompt: Rebound
      mask DialogControl text_restr_area Prompt: Restr. Area (m^2)
      mask DialogControl text_cd Prompt: Cd
      mask DialogControl cont_blowoff_prv Prompt: Blowoff PRV
      mask DialogControl text_blowoff_prv_comp Prompt: Compression
      mask DialogControl text_blowoff_prv_reb Prompt: Rebound
      mask DialogControl text_psetdiff Prompt: Press. Diff. (MPa)
      mask DialogControl text_prange Prompt: Press. Range (MPa)
      mask DialogControl text_areamax Prompt: Max Area (m^2)
      mask DialogControl text_blowoff_cd Prompt: Cd
      mask DialogControl cont_dpr_cvd_valve Prompt: CVD Valve
      mask DialogControl tab_ride_height Prompt: Ride Height
      mask DialogControl text_rideheight_inlet Prompt: Inlet
      mask DialogControl text_rideheight_outlet Prompt: Outlet
      mask DialogControl text_rh_prcv_cmpos Prompt: Orifice Pos. Vec. (m)
      mask DialogControl text_rh_prcv_orificearea Prompt: Orifice Area Vec (m^2)
      mask DialogControl text_rh_prcv_orificepdiff Prompt: Orifice Pr. Diff (bar)
      mask DialogControl text_rh_prcv_pcprange Prompt: Pr. Comp. Range (bar)
      mask DialogControl text_rh_prcv_pcamax Prompt: Pr. Comp. A Max (m^2)
      mask DialogControl text_rh_prcv_arealeak Prompt: Leakage Area (m^2)
      mask DialogControl text_rh_prcv_cd Prompt: Cd
      mask DialogControl text_rh_fcv_smooth Prompt: Smoothing
      mask DialogControl text_rh_fcv_tfilt Prompt: Time Constant (s)
  Linear : Subsystem  VariantControl=Linear  mask(Linear Spring){spr_def0=Spring.xPreload.Value, spr_frc0=Spring.fPreload.Value, spr_k=Spring.K.Value, spr_hp_top=Spring.sTop.Value, spr_hp_bot=Spring.sBottom.Value}
      mask prompts: spr_def0 "Preload Deformation (m)"; spr_frc0 "Preload Force (N)"; spr_k "Spring Rate (N/m)"; spr_hp_top "HP Top [xyz] (m)"; spr_hp_bot "HP Bottom [xyz] (m)"
      mask help: Spring with linear stiffness. Preload can be specified using deformation or force, unused value must be zero. If both are non-zero, preload deformation is used.
      mask init: same as sm_car/Vehicle/Vehicle/Chassis/Spring/Decoupled/Spring A1 Heave/Linear
      mask DialogControl Container3 Prompt: Specify Preload Deformation or Force, other value is 0
  No Spring : Subsystem  VariantControl=No_Spring  mask(No Spring){}
      mask help: Sensor only
  Nonlinear : Subsystem  VariantControl=Nonlinear  mask(Nonlinear Spring){spr_def0=Spring.xPreload.Value, spr_frc0=Spring.fPreload.Value, deformation_vector=Spring.xSpring.Value, force_vector=Spring.fSpring.Value, spr_hp_top=Spring.sTop.Value, spr_hp_bot=Spring.sBottom.Value}
      mask prompts: spr_def0 "Preload Deformation (m)"; spr_frc0 "Preload Force (N)"; deformation_vector "Deformation vector"; force_vector "Force vector"; spr_hp_top "HP Top [xyz] (m)"; spr_hp_bot "HP Bottom [xyz] (m)"
      mask help: Spring with stiffness specified by a lookup table. Preload can be specified using deformation or force, unused value must be zero. If both are non-zero, preload deformation is used.
      mask init:
      | spr_len0 = norm(spr_hp_top-spr_hp_bot);
      | 
      | curblk = gcb;
      | spr_x0 = -spr_def0;
      | if(spr_def0==0 && (abs(spr_frc0)>0))
      | spr_x0 = -interp1(force_vector,deformation_vector,spr_frc0);
      | end
      mask TypeOptions deformation_vector: Spring/deformation_vector
      mask TypeOptions force_vector: Spring/force_vector
      mask DialogControl Container3 Prompt: Specify Preload Deformation or Force, other value is 0
  " R" : PMIOPort  Side=Left
  " C" : PMIOPort  Port=2  Side=Right
  " meas" : Outport  VectorParamsAs1DForOutWhenUnconnected=off
